simulink model "Main1"  (R2022b)
settings: Solver=ode23  StartTime=0.0  StopTime=inf  MaxStep=0.00001  RelTol=1e-3
model workspace (MAT data in the model file):
  Bs = 0.0014
  Caster_Angle = 7
  Cornering_Stiffness = Simulink.Parameter
  Cornering_Stiffness.Value = 1500
  Cornering_Stiffness.DataType = 'double'
  Cornering_Stiffness.Complexity = 'real'
  Cornering_Stiffness.Dimensions = [1 1]
  Endstop_Torque = Simulink.Parameter
  Endstop_Torque.Value = 3
  Endstop_Torque.DataType = 'auto'
  Endstop_Torque.Complexity = 'real'
  Endstop_Torque.Dimensions = [1 1]
  FyL = 3600
  FyR = 3600
  Fz = 3000
  FzL = 3000
  FzR = 3000
  Js = 0.015
  K_Tire = 0.00125
  Kingpin_Angle = 14
  Lateral_Force = Simulink.Parameter
  Lateral_Force.Value = -2286.13566081
  Lateral_Force.DataType = 'auto'
  Lateral_Force.Complexity = 'real'
  Lateral_Force.Dimensions = [1 1]
  Lower_Limit_Wf = 0.2
  Mass = Simulink.Parameter
  Mass.Value = 1000
  Mass.DataType = 'auto'
  Mass.Complexity = 'real'
  Mass.Dimensions = [1 1]
  Mu = Simulink.Parameter
  Mu.Value = 0.7
  Mu.DataType = 'double'
  Mu.Complexity = 'real'
  Mu.Dimensions = [1 1]
  Rear_Slip_Angle = Simulink.Parameter
  Rear_Slip_Angle.Value = 0.5
  Rear_Slip_Angle.DataType = 'auto'
  Rear_Slip_Angle.Complexity = 'real'
  Rear_Slip_Angle.Dimensions = [1 1]
  Rolling_Radius = 0.268
  Slip_Angle = 4.73317464193
  Standard_Dev = 1
  Steer_Angle = -32.2953148908
  Var = 0
  Var1 = 0
  Vehicle_Speed = Simulink.Parameter
  Vehicle_Speed.Value = 11.9684842428
  Vehicle_Speed.DataType = 'auto'
  Vehicle_Speed.Min = 0
  Vehicle_Speed.Max = 150
  Vehicle_Speed.Complexity = 'real'
  Vehicle_Speed.Dimensions = [1 1]
  Wf = 1
  d = 0.025
  tp0 = 0.025
settings Model: Creator=AGR  LastModifiedBy=AGR

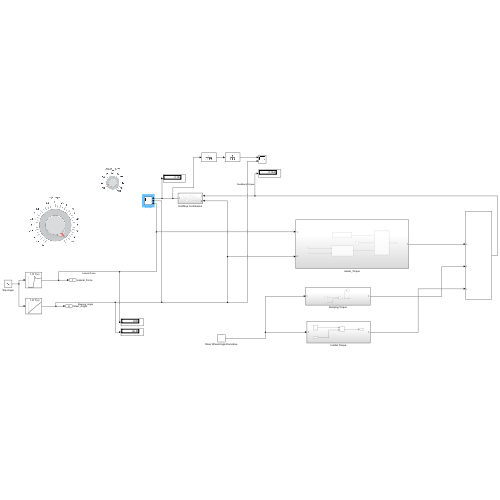
[thumbnail: Simulink's stored preview of the top-level diagram]
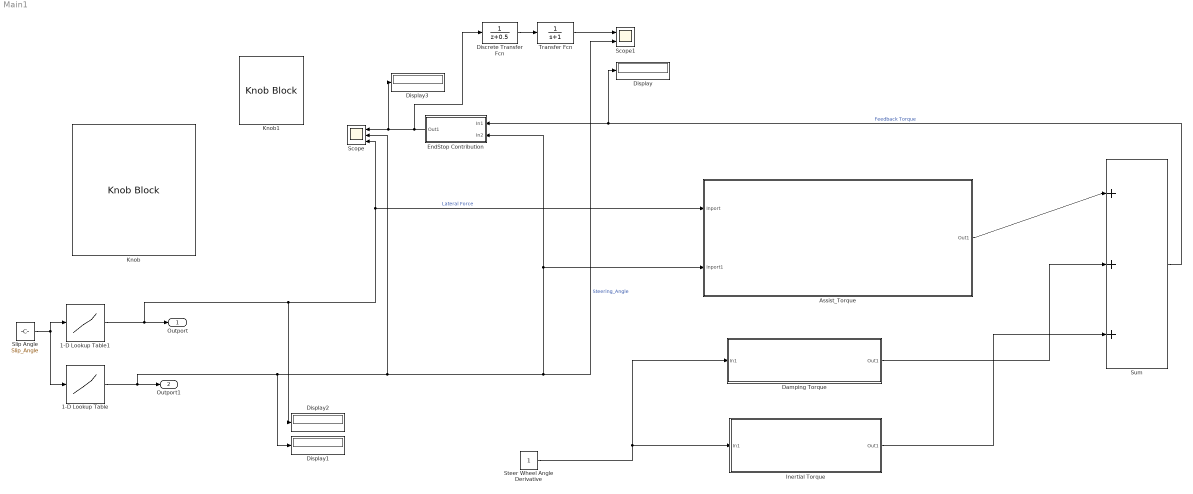
== system Main1 ==
  1-D Lookup Table : Lookup_n-D  NumberOfTableDimensions=1  BreakpointsForDimension1=[-5 -4 -3 -2 -1 0 1 2 3 4 5]  IndexSearchMethod=Linear search  Table=[-70 :14:70]  InternalRulePriority=Speed  RndMeth=Simplest
  1-D Lookup Table1 : Lookup_n-D  NumberOfTableDimensions=1  BreakpointsForDimension1=[-5:5]  Table=[-2000,-2000,-2000,-2000,-2000,3000,2000,2000,2000,2000,2000]  InternalRulePriority=Speed  RndMeth=Simplest
  Assist_Torque : Subsystem
  Damping Torque : Subsystem
  Discrete Transfer Fcn : DiscreteTransferFcn
  Display{,1..3} (4 alike) : Display
  EndStop Contribution : Subsystem
  Inertial Torque : Subsystem
  Knob : KnobBlock  ScaleMin=-5  ScaleMax=5
  Knob1 : KnobBlock
  Scope : Scope  NumInputPorts=3
  Scope1 : Scope  NumInputPorts=2
  Slip Angle : Constant  Value=Slip_Angle
  Steer Wheel Angle Derivative : Constant
  Sum : Sum  Inputs=|+++
  Transfer Fcn : TransferFcn  Denominator=[1 1]
  Outport : Outport  SignalName=Lateral_Force
  Outport1 : Outport  Port=2  SignalName=Steer_Angle
  wires:
  Assist_Torque/1(Out1) -> Sum/1
  Sum/1 -> Display/1, EndStop Contribution/1(In1)  "Feedback Torque"
  Steer Wheel Angle Derivative/1 -> Inertial Torque/1(In1), Damping Torque/1(In1)
  Slip Angle/1 -> 1-D Lookup Table/1, 1-D Lookup Table1/1
  1-D Lookup Table1/1 -> Display2/1, Scope/3, Assist_Torque/1(Inport), Outport/1  "Lateral Force"
  1-D Lookup Table/1 -> Scope1/2, Assist_Torque/2(Inport1), EndStop Contribution/2(In2), Scope/2, Display1/1, Outport1/1  "Steering_Angle"
  Inertial Torque/1(Out1) -> Sum/3
  Damping Torque/1(Out1) -> Sum/2
  EndStop Contribution/1(Out1) -> Discrete Transfer Fcn/1, Display3/1, Scope/1
  Discrete Transfer Fcn/1 -> Transfer Fcn/1
  Transfer Fcn/1 -> Scope1/1

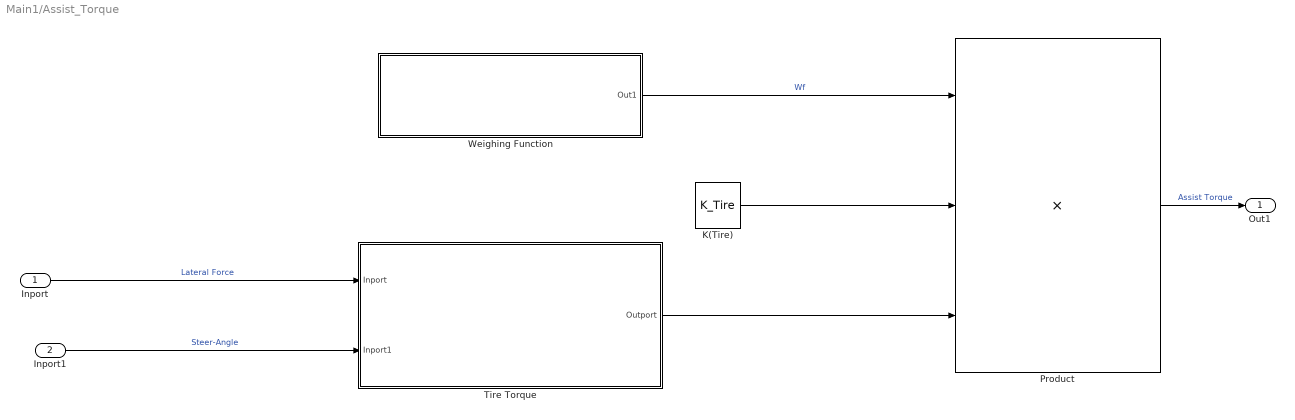
== system Main1/Assist_Torque ==
  Inport : Inport
  Inport1 : Inport  Port=2
  K(Tire) : Constant  Value=K_Tire
  Product : Product  Inputs=3
  Tire Torque : Subsystem
  Weighing Function : Subsystem
  Out1 : Outport
  wires:
  Tire Torque/1(Outport) -> Product/3
  K(Tire)/1 -> Product/2
  Weighing Function/1(Out1) -> Product/1  "Wf"
  Product/1 -> Out1/1  "Assist Torque"
  Inport/1 -> Tire Torque/1(Inport)  "Lateral Force"
  Inport1/1 -> Tire Torque/2(Inport1)  "Steer-Angle"

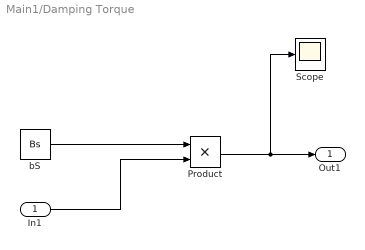
== system Main1/Damping Torque ==
  In1 : Inport
  Product : Product
  Scope : Scope
  bS : Constant  Value=Bs  SampleTime=1
  Out1 : Outport
  wires:
  bS/1 -> Product/1
  In1/1 -> Product/2
  Product/1 -> Scope/1, Out1/1

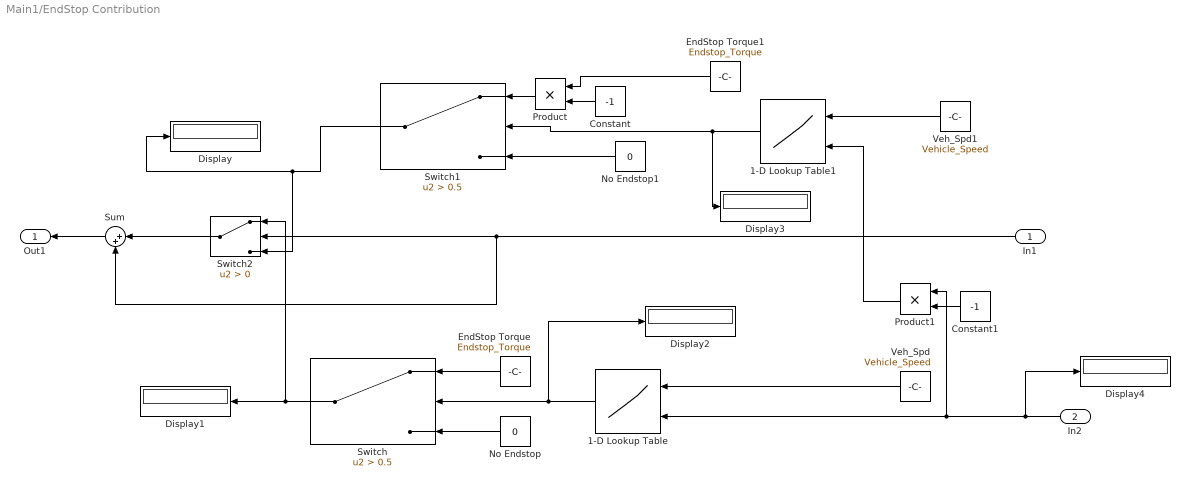
== system Main1/EndStop Contribution ==
  In1 : Inport
  In2 : Inport  Port=2
  1-D Lookup Table : Lookup_n-D  BreakpointsForDimension1=[0 20 40 60 80]  BreakpointsForDimension2=[-70 -65 -60 -55 -50]  Table=[1 0 0 0 0;0 1 0 0 0;0 0 1 0 0;0 0 0 1 0;0 0 0 0 1]  InternalRulePriority=Speed  RndMeth=Simplest
      settings: InputPortMap=u0,u1
  1-D Lookup Table1 : Lookup_n-D  BreakpointsForDimension1=[0 20 40 60 80]  BreakpointsForDimension2=[-70 -65 -60 -55 -50]  Table=[1 0 0 0 0;0 1 0 0 0;0 0 1 0 0;0 0 0 1 0;0 0 0 0 1]  InternalRulePriority=Speed  RndMeth=Simplest
      settings: InputPortMap=u0,u1
  Constant : Constant  Value=-1
  Constant1 : Constant  Value=-1
  Display{,1..4} (5 alike) : Display
  EndStop Torque : Constant  Value=Endstop_Torque
  EndStop Torque1 : Constant  Value=Endstop_Torque
  No Endstop : Constant  Value=0
  No Endstop1 : Constant  Value=0
  Product : Product
  Product1 : Product
  Sum : Sum  Inputs=|++
  Switch : Switch  Criteria=u2 > Threshold  Threshold=0.5  SaturateOnIntegerOverflow=off  InputSameDT=off
  Switch1 : Switch  Criteria=u2 > Threshold  Threshold=0.5  SaturateOnIntegerOverflow=off  InputSameDT=off
  Switch2 : Switch  Criteria=u2 > Threshold  SaturateOnIntegerOverflow=off  InputSameDT=off
  Veh_Spd : Constant  Value=Vehicle_Speed
  Veh_Spd1 : Constant  Value=Vehicle_Speed
  Out1 : Outport
  wires:
  EndStop Torque/1 -> Switch/1
  No Endstop/1 -> Switch/3
  Veh_Spd/1 -> 1-D Lookup Table/1
  1-D Lookup Table/1 -> Display2/1, Switch/2
  1-D Lookup Table1/1 -> Display3/1, Switch1/2
  Veh_Spd1/1 -> 1-D Lookup Table1/1
  In2/1 -> Display4/1, Product1/1, 1-D Lookup Table/2
  No Endstop1/1 -> Switch1/3
  Product/1 -> Switch1/1
  EndStop Torque1/1 -> Product/1
  Constant/1 -> Product/2
  In1/1 -> Switch2/2, Sum/2
  Switch1/1 -> Switch2/3, Display/1
  Switch/1 -> Switch2/1, Display1/1
  Constant1/1 -> Product1/2
  Product1/1 -> 1-D Lookup Table1/2
  Switch2/1 -> Sum/1
  Sum/1 -> Out1/1

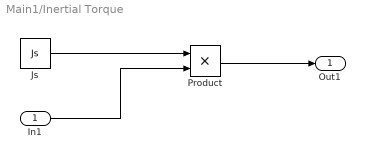
== system Main1/Inertial Torque ==
  In1 : Inport
  Js : Constant  Value=Js  SampleTime=1
  Product : Product
  Out1 : Outport
  wires:
  Js/1 -> Product/1
  Product/1 -> Out1/1
  In1/1 -> Product/2

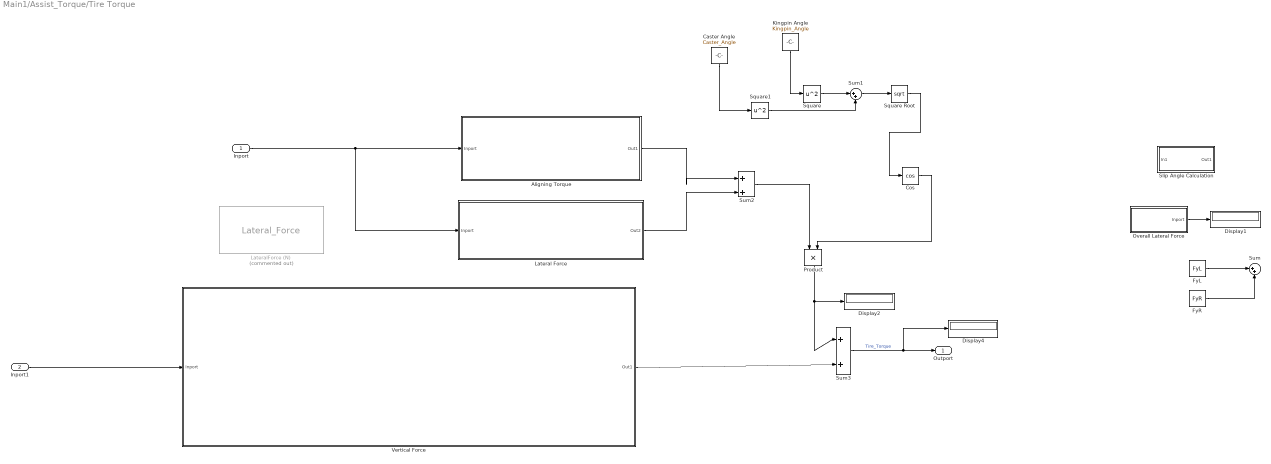
== system Main1/Assist_Torque/Tire Torque ==
  Inport : Inport
  Inport1 : Inport  Port=2
  Aligning Torque : Subsystem
  "Caster Angle " : Constant  Value=Caster_Angle  LockScale=on
  Cos : Trigonometry  Operator=cos
  Display1 : Display
  Display2 : Display
  Display4 : Display
  FyL : Constant  Value=FyL
  FyR : Constant  Value=FyR
  Kingpin Angle : Constant  Value=Kingpin_Angle
  Lateral Force : Subsystem
  LateralForce (N) : Constant  Commented=on  Value=Lateral_Force
  Overall Lateral Force : Subsystem
  Product : Product
  Slip Angle Calculation : Subsystem
  Square : Math  Operator=square  SignedPower=on  RndMeth=Zero
  Square Root : Sqrt
  Square1 : Math  Operator=square  SignedPower=on  RndMeth=Zero
  Sum{,1..3} (4 alike) : Sum  Inputs=|++
  Vertical Force : Subsystem
  Outport : Outport
  wires:
  Aligning Torque/1(Out1) -> Sum2/1
  Lateral Force/1(Out2) -> Sum2/2
  "Caster Angle "/1 -> Square1/1
  Kingpin Angle/1 -> Square/1
  Square/1 -> Sum1/1
  Square1/1 -> Sum1/2
  Sum1/1 -> Square Root/1
  Sum2/1 -> Product/1
  Square Root/1 -> Cos/1
  Vertical Force/1(Out1) -> Sum3/2
  Sum3/1 -> Display4/1, Outport/1  "Tire_Torque"
  Product/1 -> Display2/1, Sum3/1
  Cos/1 -> Product/2
  FyL/1 -> Sum/1
  Overall Lateral Force/1(Inport) -> Display1/1
  FyR/1 -> Sum/2
  Inport/1 -> Lateral Force/1(Inport), Aligning Torque/1(Inport)
  Inport1/1 -> Vertical Force/1(Inport)

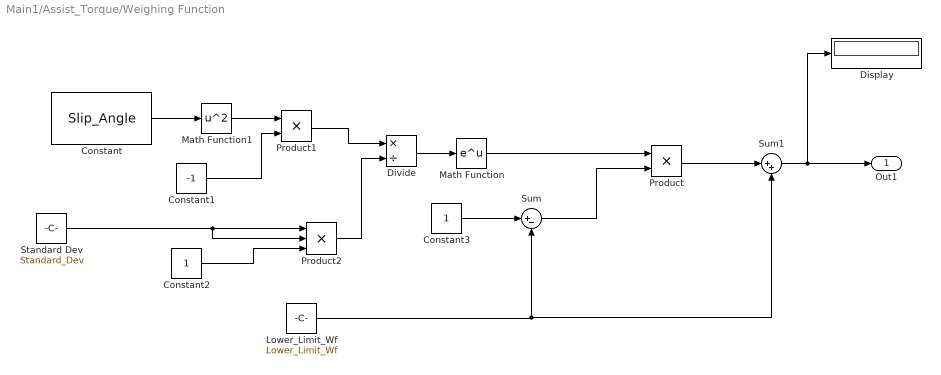
== system Main1/Assist_Torque/Weighing Function ==
  Constant : Constant  Value=Slip_Angle  SampleTime=-1
  Constant1 : Constant  Value=-1
  Constant2 : Constant
  Constant3 : Constant
  Display : Display
  Divide : Product  Inputs=*/
  Lower_Limit_Wf : Constant  Value=Lower_Limit_Wf
  Math Function : Math
  Math Function1 : Math  Operator=square
  Product : Product
  Product1 : Product
  Product2 : Product  Inputs=3
  Standard Dev : Constant  Value=Standard_Dev  VectorParams1D=off
  Sum : Sum  Inputs=|+-
  Sum1 : Sum  Inputs=|++
  Out1 : Outport
  wires:
  Standard Dev/1 -> Product2/2, Product2/1
  Constant2/1 -> Product2/3
  Product2/1 -> Divide/2
  Constant1/1 -> Product1/2
  Constant/1 -> Math Function1/1
  Math Function1/1 -> Product1/1
  Divide/1 -> Math Function/1
  Product1/1 -> Divide/1
  Math Function/1 -> Product/1
  Constant3/1 -> Sum/1
  Lower_Limit_Wf/1 -> Sum1/2, Sum/2
  Sum/1 -> Product/2
  Product/1 -> Sum1/1
  Sum1/1 -> Out1/1, Display/1

== system Main1/Assist_Torque/Tire Torque/Aligning Torque ==
  Inport : Inport
  Pneumatic Trial Estimation : Subsystem
  Product : Product
  Out1 : Outport
  wires:
  Pneumatic Trial Estimation/1(tp) -> Product/1  "tp"
  Product/1 -> Out1/1  "MA"
  Inport/1 -> Product/2

== system Main1/Assist_Torque/Tire Torque/Lateral Force ==
  Inport : Inport
  Mechanical Trial computation : Subsystem
  Product1 : Product
  Out2 : Outport
  wires:
  Mechanical Trial computation/1(Out2) -> Product1/2  "tm"
  Product1/1 -> Out2/1  "ML"
  Inport/1 -> Product1/1

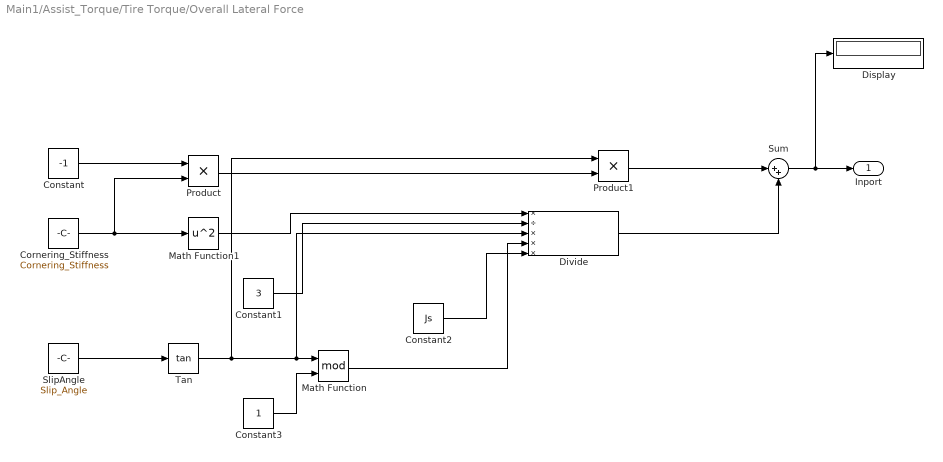
== system Main1/Assist_Torque/Tire Torque/Overall Lateral Force ==
  Constant : Constant  Value=-1
  Constant1 : Constant  Value=3
  Constant2 : Constant  Value=Js
  Constant3 : Constant
  Cornering_Stiffness : Constant  Value=Cornering_Stiffness  SampleTime=-1
  Display : Display
  Divide : Product  Inputs=*/***
  Math Function : Math  Operator=mod
  Math Function1 : Math  Operator=square
  Product : Product
  Product1 : Product
  SlipAngle : Constant  Value=Slip_Angle  SampleTime=-1
  Sum : Sum  Inputs=|++
  Tan : Trigonometry  Operator=tan
  Inport : Outport
  wires:
  SlipAngle/1 -> Tan/1
  Tan/1 -> Product1/1, Math Function/1, Divide/3
  Cornering_Stiffness/1 -> Product/2, Math Function1/1
  Constant/1 -> Product/1
  Math Function1/1 -> Divide/1
  Constant1/1 -> Divide/2
  Constant2/1 -> Divide/5
  Product/1 -> Product1/2
  Product1/1 -> Sum/1
  Divide/1 -> Sum/2
  Sum/1 -> Display/1, Inport/1
  Constant3/1 -> Math Function/2
  Math Function/1 -> Divide/4

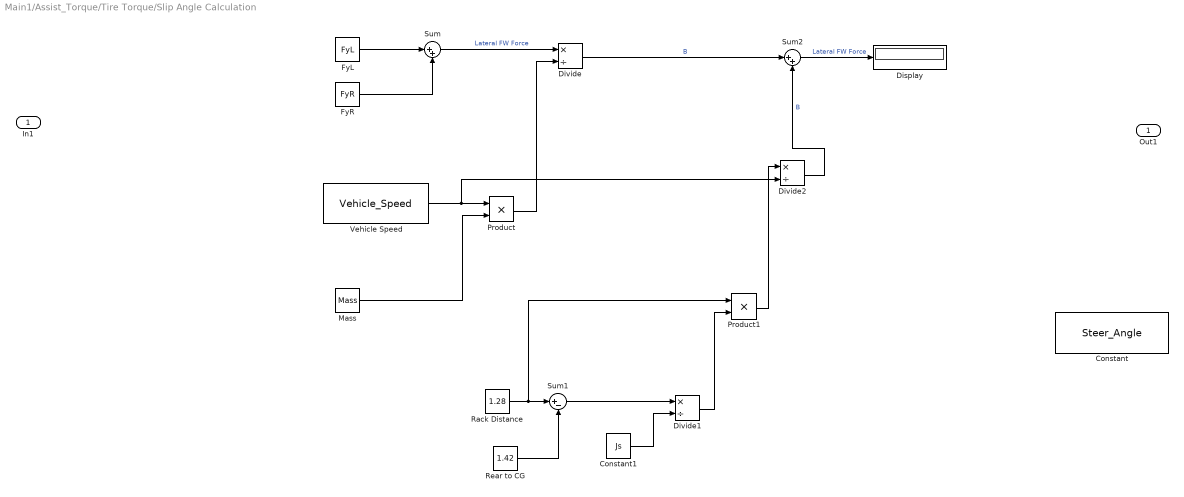
== system Main1/Assist_Torque/Tire Torque/Slip Angle Calculation ==
  In1 : Inport
  Constant : Constant  Value=Steer_Angle
  Constant1 : Constant  Value=Js
  Display : Display
  Divide : Product  Inputs=*/
  Divide1 : Product  Inputs=*/
  Divide2 : Product  Inputs=*/
  FyL : Constant  Value=FyL
  FyR : Constant  Value=FyR
  Mass : Constant  Value=Mass
  Product : Product
  Product1 : Product
  Rack Distance : Constant  Value=1.28
  Rear to CG : Constant  Value=1.42
  Sum : Sum  Inputs=|++
  Sum1 : Sum  Inputs=|+-
  Sum2 : Sum  Inputs=|++
  Vehicle Speed : Constant  Value=Vehicle_Speed
  Out1 : Outport
  wires:
  Sum/1 -> Divide/1  "Lateral FW Force"
  FyL/1 -> Sum/1
  FyR/1 -> Sum/2
  Product/1 -> Divide/2
  Vehicle Speed/1 -> Divide2/2, Product/1
  Mass/1 -> Product/2
  Divide/1 -> Sum2/1  "B"
  Divide1/1 -> Product1/2
  Sum1/1 -> Divide1/1
  Rear to CG/1 -> Sum1/2
  Rack Distance/1 -> Product1/1, Sum1/1
  Constant1/1 -> Divide1/2
  Product1/1 -> Divide2/1
  Divide2/1 -> Sum2/2  "B"
  Sum2/1 -> Display/1  "Lateral FW Force"

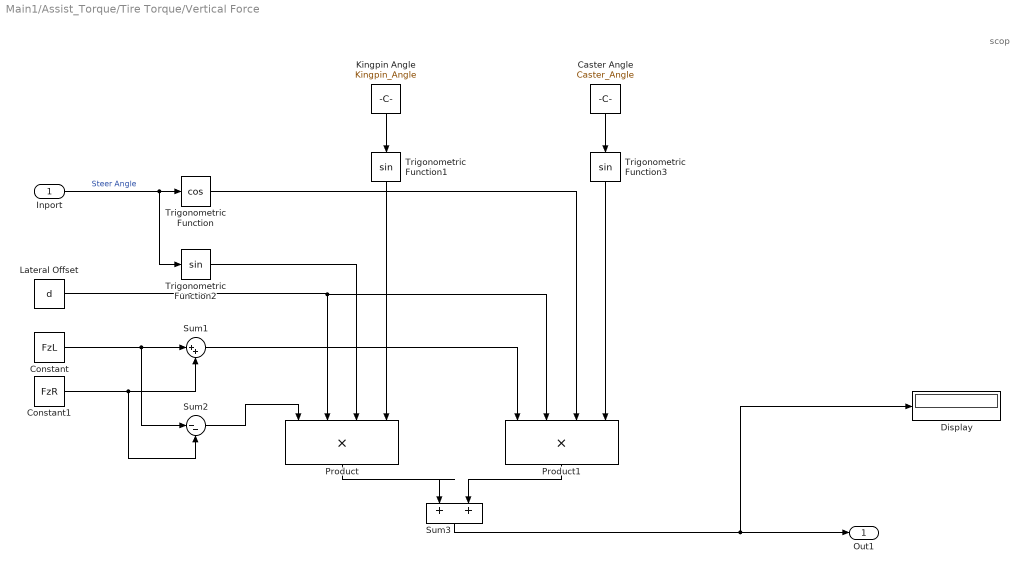
== system Main1/Assist_Torque/Tire Torque/Vertical Force ==
  note: scop
  Inport : Inport
  "Caster Angle " : Constant  Value=Caster_Angle  LockScale=on
  Constant : Constant  Value=FzL
  Constant1 : Constant  Value=FzR
  Display : Display
  Kingpin Angle : Constant  Value=Kingpin_Angle
  Lateral Offset : Constant  Value=d
  Product : Product  Inputs=4
  Product1 : Product  Inputs=4
  Sum1 : Sum  Inputs=|++
  Sum2 : Sum  Inputs=|--
  Sum3 : Sum  Inputs=|++
  Trigonometric Function : Trigonometry  Operator=cos
  Trigonometric Function1 : Trigonometry
  Trigonometric Function2 : Trigonometry
  Trigonometric Function3 : Trigonometry
  Out1 : Outport
  wires:
  Trigonometric Function3/1 -> Product1/4
  Trigonometric Function/1 -> Product1/3
  Trigonometric Function2/1 -> Product/3
  Inport/1 -> Trigonometric Function/1, Trigonometric Function2/1  "Steer Angle"
  Kingpin Angle/1 -> Trigonometric Function1/1
  Sum3/1 -> Display/1, Out1/1
  Sum1/1 -> Product1/1
  Constant/1 -> Sum2/1, Sum1/1
  "Caster Angle "/1 -> Trigonometric Function3/1
  Constant1/1 -> Sum2/2, Sum1/2
  Lateral Offset/1 -> Product1/2, Product/2
  Product1/1 -> Sum3/2
  Product/1 -> Sum3/1
  Sum2/1 -> Product/1
  Trigonometric Function1/1 -> Product/4

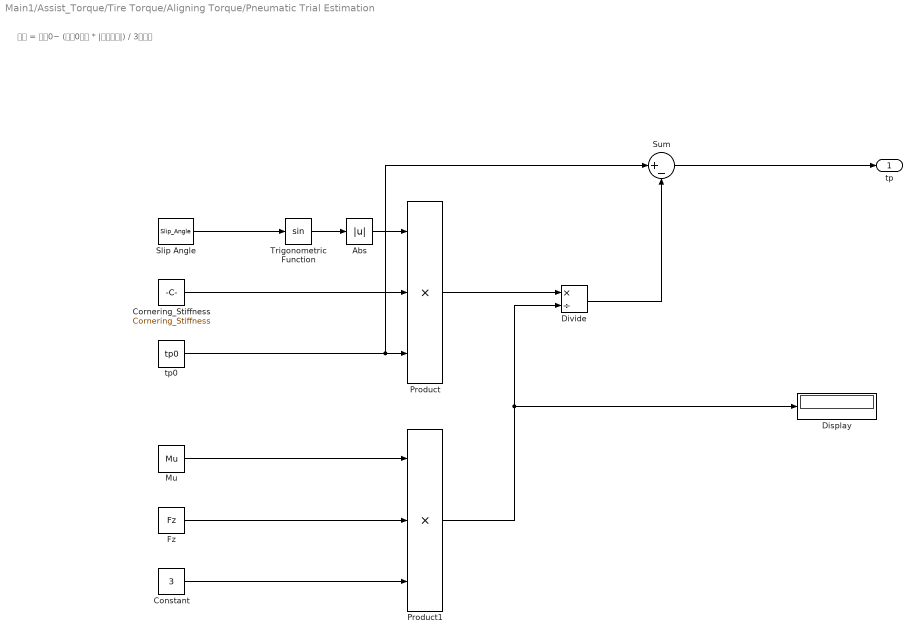
== system Main1/Assist_Torque/Tire Torque/Aligning Torque/Pneumatic Trial Estimation ==
  note: 𝑡𝑝 = 𝑡𝑝0− (𝑡𝑝0𝐶𝛼 * |𝑡𝑎𝑛𝛼|) / 3𝜇𝐹𝑍
  Abs : Abs  SaturateOnIntegerOverflow=off
  Constant : Constant  Value=3
  Cornering_Stiffness : Constant  Value=Cornering_Stiffness
  Display : Display
  Divide : Product  Inputs=*/
  Fz : Constant  Value=Fz
  Mu : Constant  Value=Mu  VectorParams1D=off
  Product : Product  Inputs=3
  Product1 : Product  Inputs=3
  Slip Angle : Constant  Value=Slip_Angle  SampleTime=1
  Sum : Sum  Inputs=|+-
  Trigonometric Function : Trigonometry
  tp0 : Constant  Value=tp0
  tp : Outport
  wires:
  Cornering_Stiffness/1 -> Product/2
  tp0/1 -> Sum/1, Product/3
  Abs/1 -> Product/1
  Slip Angle/1 -> Trigonometric Function/1
  Trigonometric Function/1 -> Abs/1
  Product/1 -> Divide/1
  Mu/1 -> Product1/1
  Fz/1 -> Product1/2
  Constant/1 -> Product1/3
  Product1/1 -> Display/1, Divide/2
  Divide/1 -> Sum/2
  Sum/1 -> tp/1

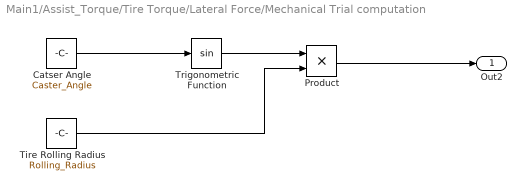
== system Main1/Assist_Torque/Tire Torque/Lateral Force/Mechanical Trial computation ==
  "Catser Angle " : Constant  Value=Caster_Angle  LockScale=on
  Product : Product
  Tire Rolling Radius : Constant  Value=Rolling_Radius
  Trigonometric Function : Trigonometry
  Out2 : Outport
  wires:
  "Catser Angle "/1 -> Trigonometric Function/1
  Trigonometric Function/1 -> Product/1
  Tire Rolling Radius/1 -> Product/2
  Product/1 -> Out2/1
